simulink model "num2ASCIIsequenced"  (Simulink 7.3)
settings: Solver=FixedStepDiscrete  StartTime=0.0  StopTime=.1  FixedStep=.0005  RelTol=1e-3
libraries: dsPICdrivers x9, simulink x3
settings Model: Creator=ij8977  LastModifiedBy=ij8977  ExtModeTrigDuration=10000
settings SolverCC: PositivePriorityOrder=on
settings OptimizationCC: OptimizeModelRefInitCode=on  LifeSpan=1
settings HardwareCC: ProdBitPerInt=16  ProdEndianess=LittleEndian  ProdWordSize=16  ProdHWDeviceType=16-bit Generic
settings RTWCC: SystemTargetFile=dspic.tlc  TemplateMakefile=dspic_pic30_gcc.tmf  PostCodeGenCommand=dsPIC_Compile()  Description=Embedded Target for Microchip dsPIC (real-time)  ProcessScript=dspic_make_rtw_hook
settings CodeAppCC: IgnoreCustomStorageClasses=off
settings STFCustomTargetCC: ModelReferenceCompliant=off  IncludeMdlTerminateFcn=off  CombineOutputUpdateFcns=on  SuppressErrorStatus=on  ERTCustomFileBanners=on  SupportContinuousTime=off  SupportNonInlinedSFcns=off  SystemTargetFile=dspic.tlc
settings ERTTargetCC: MultiwordLength=2048  ModelReferenceCompliant=off  ParMdlRefBuildCompliant=off  CompOptLevelCompliant=off  IncludeMdlTerminateFcn=off  SuppressErrorStatus=on  ERTFirstTimeCompliant=off  ModelStepFunctionPrototypeControlCompliant=off  CPPClassGenCompliant=off  ExtModeMexFile=noextcomm  InlinedParameterPlacement=NonHierarchical  ERTSrcFileBannerTemplate=dsPIC_code_template.cgt  ERTHdrFileBannerTemplate=dsPIC_code_template.cgt  ERTDataSrcFileTemplate=dsPIC_code_template.cgt  ERTDataHdrFileTemplate=dsPIC_code_template.cgt  ERTCustomFileTemplate=dsPIC_main.tlc
settings CustomProperty: DataType=string  Value=C:\PROGRA~1\MATLAB\R2009a\bin\win32\gmake

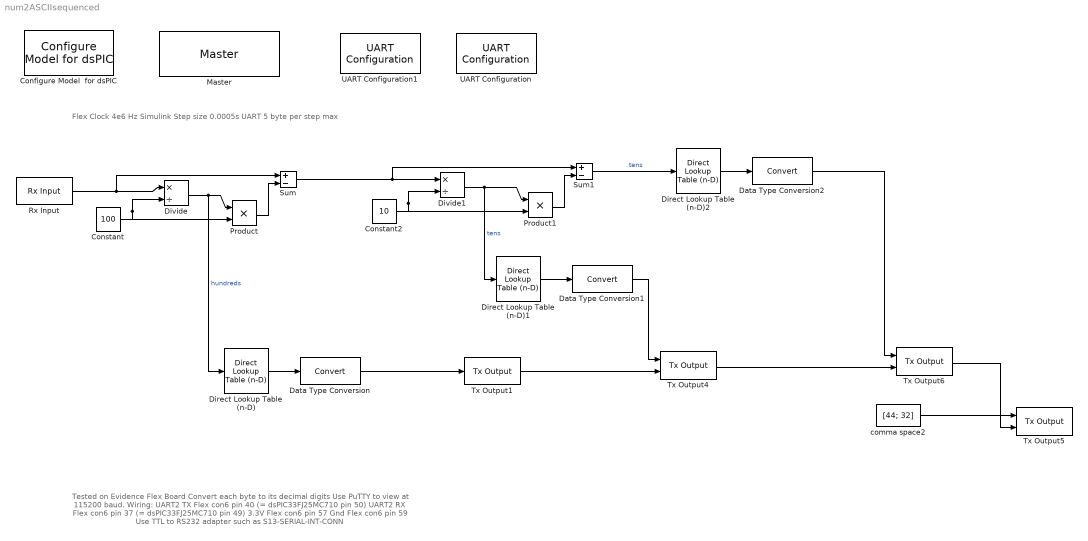
== system num2ASCIIsequenced ==
  note: Tested on Evidence Flex Board
      | Convert each byte to its decimal digits
      | Use PuTTY to view at 115200 baud.
      |
      | Wiring:
      | UART2 TX Flex con6 pin 40 (= dsPIC33FJ25MC710 pin 50)
      | UART2 RX Flex con6 pin 37 (= dsPIC33FJ25MC710 pin 49)
      | 3.3V Flex con6 pin 57
      | Gnd Flex con6 pin 59
      |
      | Use TTL to RS232 adapter such as S13-SERIAL-INT-CONN
  note: Flex Clock 4e6 Hz
      | Simulink Step size 0.0005s
      | UART 5 byte per step max
  Configure Model  for dsPIC : dsPICdrivers/Simulink Configuration/Configure Model  for dsPIC
  Constant : Constant  Value=100  OutDataType=fixdt(1, 16)  OutScaling=2^0
  Constant2 : Constant  Value=10  OutDataType=fixdt(1, 16)  OutScaling=2^0
  Data Type Conversion : DataTypeConversion  OutDataType=fixdt(1, 16)  OutScaling=2^0
  Data Type Conversion1 : DataTypeConversion  OutDataType=fixdt(1, 16)  OutScaling=2^0
  Data Type Conversion2 : DataTypeConversion  OutDataType=fixdt(1, 16)  OutScaling=2^0
  Direct Lookup Table (n-D) : simulink/Lookup Tables/Direct Lookup Table (n-D)  maskTabDims=1  explicitNumDims=1  outDims=Element  tabIsInput=off  mxTable=[48;49;50;51;52;53;54;55;56;57]  clipFlag=Warning  samptime=-1
  Direct Lookup Table (n-D)1 : simulink/Lookup Tables/Direct Lookup Table (n-D)  maskTabDims=1  explicitNumDims=1  outDims=Element  tabIsInput=off  mxTable=[48;49;50;51;52;53;54;55;56;57]  clipFlag=Warning  samptime=-1
  Direct Lookup Table (n-D)2 : simulink/Lookup Tables/Direct Lookup Table (n-D)  maskTabDims=1  explicitNumDims=1  outDims=Element  tabIsInput=off  mxTable=[48;49;50;51;52;53;54;55;56;57]  clipFlag=Warning  samptime=-1
  Divide : Product  Inputs=*/  OutDataTypeMode=uint8  OutDataType=fixdt(1, 16)  OutScaling=2^-10  OutDataTypeStr=uint8
  Divide1 : Product  Inputs=*/  OutDataTypeMode=uint8  OutDataType=fixdt(1, 16)  OutScaling=2^-10  OutDataTypeStr=uint8
  Master : dsPICdrivers/Master  Tag=dsPIC_MASTER  Priority=1  TimeStepType=Timer1  picType=33fJ256MC710  fcy=40000000  Quartz_33f=4e6  PLLActive_33f=on  fcyDesired_33f=40000000  tmr1="[1  19999  0]"  tmr1Info="Time Step : 0.0005  ;   Error : 0%  PR1=19999"  tmr2345="[0  0  0  0  0  0  0  0]"  tmr2345cfg=[-1 -1 -1 -1 -1 -1 -1 -1]  IOautoConf=on  typePort="[ 0  0  0  0  0  0  0  0  0  0  0  0  0  0  0  0  0  0  0  0  0  0  0  0  0  0  0  0  0  0  0  0  0  0  0  0  0  0  0  0  0  0  0  0  0  0  0  0  0  0  0  0  0  0  0  0  0  0  0  0  0  0  0  0  0  0  0  0  0  0  0  0  0  0  0  0  0  0  0  0  0  0  4  0  4  5  0  0  0  0  0  0  0  0  0  0  0  0  0  0  0  0  0  0  0  0  0  0  0  0  0  0 ]"  TRIS="[ 65535  65535  65535  65535  65535  65535  65535 ]"  ADPCFG=0  MasterBusyPort=None  MasterOverloadPort=None  FOSC=Quartz (XT - HS)  ClockSwitchMonitor=Both disabled  TempProtection_33f=TEMP_ON  FPBOR=<empty>  PWRT=disable  MCLR=<empty>  PowerSave=off  OverrideFcy=off  NewFcy=1e6  PR2345="[65535  65535  65535  65535  65535  65535  65535  65535]"
  Product : Product  OutDataType=fixdt(1, 16)  OutScaling=2^0  RndMeth=Zero
  Product1 : Product  OutDataType=fixdt(1, 16)  OutScaling=2^0  RndMeth=Zero
  Rx Input : dsPICdrivers/Serial PORT/Rx Input  Tag=dsPIC_RX  Priority=5  UART=1  SampleTime=-1  BlockingFctChk=off  OutputDefault=0  IsPresentFlagChk=off
  Sum : Sum  Inputs=+-  OutDataType=fixdt(1, 16)  OutScaling=2^0
  Sum1 : Sum  Inputs=+-  OutDataType=fixdt(1, 16)  OutScaling=2^0
  Tx Output1 : dsPICdrivers/Serial PORT/Tx Output  Tag=dsPIC_TX  Priority=5  UART=2  OrderingInOutPopup=Output
  Tx Output4 : dsPICdrivers/Serial PORT/Tx Output  Tag=dsPIC_TX  Priority=5  UART=2  OrderingInOutPopup=Input & Output
  Tx Output5 : dsPICdrivers/Serial PORT/Tx Output  Tag=dsPIC_TX  Priority=5  UART=2  OrderingInOutPopup=Input
  Tx Output6 : dsPICdrivers/Serial PORT/Tx Output  Tag=dsPIC_TX  Priority=5  UART=2  OrderingInOutPopup=Input & Output
  UART Configuration : dsPICdrivers/Serial PORT/UART Configuration  Tag=dsPIC_config_UART  Priority=2  UART=2  proposed_BAUD=115200  ALT_TX_RX=on  InterruptTxWhen=When Transmit Buffer is empty  TXInterruptPri=1  TxBufferSize=32  TXEN=on  InterruptRxWhen=When Receive Buffer is full (contain 4 characters)  RXInterruptPri=2  RxBufferSize=32  BAUD=115200  UxBRG=21  Info="UxBRG = 21   ||  Real Baud : 113636   ||  % error : -1.3573  ||  max 5.6818 Bytes / Step"  RealBaud=0
  UART Configuration1 : dsPICdrivers/Serial PORT/UART Configuration  Tag=dsPIC_config_UART  Priority=2  UART=1  proposed_BAUD=115200  ALT_TX_RX=on  InterruptTxWhen=When Transmit Buffer is empty  TXInterruptPri=1  TxBufferSize=32  TXEN=off  InterruptRxWhen=When Receive Buffer is full (contain 4 characters)  RXInterruptPri=2  RxBufferSize=32  BAUD=115200  UxBRG=21  Info="UxBRG = 21   ||  Real Baud : 113636   ||  % error : -1.3573  ||  max 5.6818 Bytes / Step"  RealBaud=0
  comma space2 : Constant  Value=[44; 32]  OutDataTypeMode=uint8  OutDataType=fixdt(1, 16)  OutScaling=2^0  OutDataTypeStr=uint8
  wires:
  Direct Lookup Table (n-D)/1 -> Data Type Conversion/1
  Rx Input/1 -> Divide/1, Sum/1
  Constant/1 -> Divide/2, Product/2
  Divide/1 -> Product/1, Direct Lookup Table (n-D)/1  "hundreds"
  Product/1 -> Sum/2
  Sum/1 -> Sum1/1, Divide1/1
  Constant2/1 -> Product1/2, Divide1/2
  Divide1/1 -> Product1/1, Direct Lookup Table (n-D)1/1  "tens"
  Product1/1 -> Sum1/2
  Sum1/1 -> Direct Lookup Table (n-D)2/1  "tens"
  Direct Lookup Table (n-D)1/1 -> Data Type Conversion1/1
  Direct Lookup Table (n-D)2/1 -> Data Type Conversion2/1
  Data Type Conversion2/1 -> Tx Output6/1
  Data Type Conversion/1 -> Tx Output1/1
  Data Type Conversion1/1 -> Tx Output4/1
  Tx Output1/1 -> Tx Output4/2
  Tx Output4/1 -> Tx Output6/2
  comma space2/1 -> Tx Output5/1
  Tx Output6/1 -> Tx Output5/2
